simulink model "Chapter7"  (R2024b)
settings: Solver=ode4  StartTime=0.0  StopTime=SIM.StopTime  FixedStep=SIM.FixedStepSize  RelTol=1e-3
values from neighbouring files (symbols this model uses):
  AP = computeAutopilotGains(MAV, TRIM, TFS, DES)    [ch7_main.m]
  CMD = struct()    [ch7_main.m]
  DES = loadDesignParams()    [ch7_main.m]
  LIM = loadSafetyLimits()    [ch7_main.m]
  SNS = loadSensorParameters()    [ch7_main.m]    (also in loadSensorParameters.m = struct())
  TRIM = findTrim(TRIM_MODEL, Va_trim, R_trim, gamma_trim, TRIM_DATA_FILE)    [ch7_main.m]
  WIND = loadWindParameters()    [ch7_main.m]
undefined symbols (not defined in the file or in its folder): DiscIntNeverNeededParam, drawAircraft, F, Light, MAV, MIL, plotter, SIM
libraries: simulink x19, matrix_library x2, aerolibwind2 x1
(part 2 of 2)

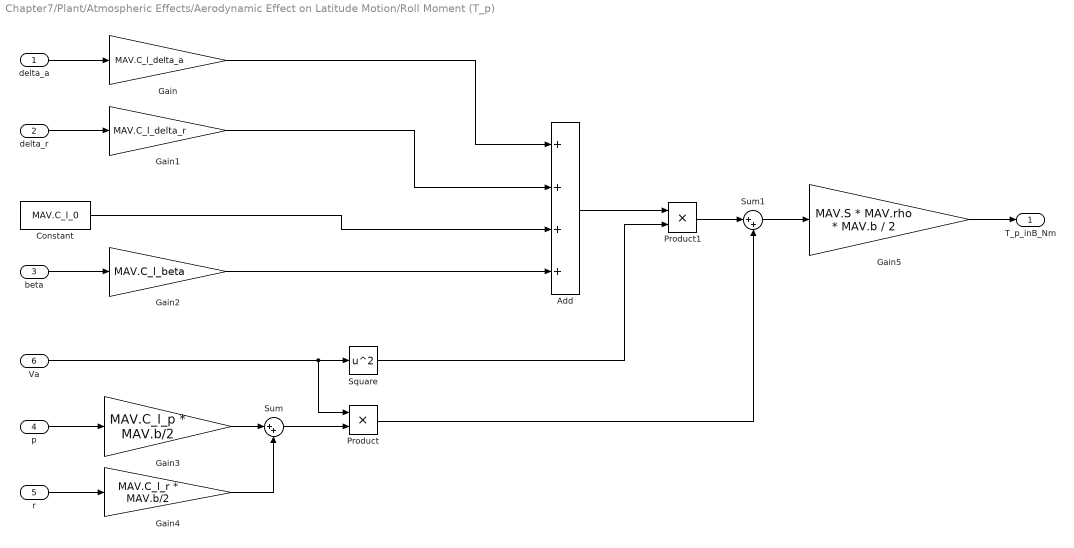
== system Chapter7/Plant/Atmospheric Effects/Aerodynamic Effect on Latitude Motion/Roll Moment (T_p) ==
  delta_a : Inport
  delta_r : Inport  Port=2
  beta : Inport  Port=3
  p : Inport  Port=4
  r : Inport  Port=5
  Va : Inport  Port=6
  Add : Sum  Inputs=++++
  Constant : Constant  Value=MAV.C_l_0
  Gain : Gain  Gain=MAV.C_l_delta_a
  Gain1 : Gain  Gain=MAV.C_l_delta_r
  Gain2 : Gain  Gain=MAV.C_l_beta
  Gain3 : Gain  Gain=MAV.C_l_p * MAV.b/2
  Gain4 : Gain  Gain=MAV.C_l_r * MAV.b/2
  Gain5 : Gain  Gain=MAV.S * MAV.rho * MAV.b / 2
  Product : Product
  Product1 : Product
  Square : Math  Operator=square
  Sum : Sum  Inputs=|++
  Sum1 : Sum  Inputs=|++
  T_p_inB_Nm : Outport
  wires:
  Gain1/1 -> Add/2
  Gain/1 -> Add/1
  Va/1 -> Square/1, Product/1
  Sum/1 -> Product/2
  Gain4/1 -> Sum/2
  Gain3/1 -> Sum/1
  r/1 -> Gain4/1
  p/1 -> Gain3/1
  Gain2/1 -> Add/4
  beta/1 -> Gain2/1
  Constant/1 -> Add/3
  delta_r/1 -> Gain1/1
  delta_a/1 -> Gain/1
  Add/1 -> Product1/1
  Square/1 -> Product1/2
  Product1/1 -> Sum1/1
  Product/1 -> Sum1/2
  Sum1/1 -> Gain5/1
  Gain5/1 -> T_p_inB_Nm/1

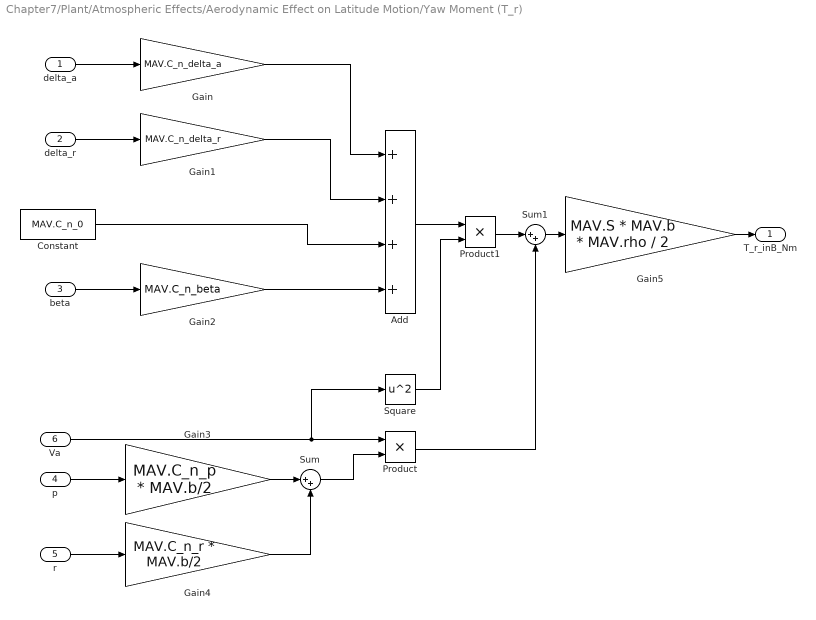
== system Chapter7/Plant/Atmospheric Effects/Aerodynamic Effect on Latitude Motion/Yaw Moment (T_r) ==
  delta_a : Inport
  delta_r : Inport  Port=2
  beta : Inport  Port=3
  p : Inport  Port=4
  r : Inport  Port=5
  Va : Inport  Port=6
  Add : Sum  Inputs=++++
  Constant : Constant  Value=MAV.C_n_0
  Gain : Gain  Gain=MAV.C_n_delta_a
  Gain1 : Gain  Gain=MAV.C_n_delta_r
  Gain2 : Gain  Gain=MAV.C_n_beta
  Gain3 : Gain  Gain=MAV.C_n_p * MAV.b/2
  Gain4 : Gain  Gain=MAV.C_n_r * MAV.b/2
  Gain5 : Gain  Gain=MAV.S * MAV.b * MAV.rho / 2
  Product : Product
  Product1 : Product
  Square : Math  Operator=square
  Sum : Sum  Inputs=|++
  Sum1 : Sum  Inputs=|++
  T_r_inB_Nm : Outport
  wires:
  Gain2/1 -> Add/4
  Constant/1 -> Add/3
  Gain1/1 -> Add/2
  delta_a/1 -> Gain/1
  p/1 -> Gain3/1
  Sum/1 -> Product/2
  Gain/1 -> Add/1
  r/1 -> Gain4/1
  Va/1 -> Square/1, Product/1
  Gain3/1 -> Sum/1
  delta_r/1 -> Gain1/1
  beta/1 -> Gain2/1
  Gain4/1 -> Sum/2
  Add/1 -> Product1/1
  Square/1 -> Product1/2
  Product1/1 -> Sum1/1
  Product/1 -> Sum1/2
  Sum1/1 -> Gain5/1
  Gain5/1 -> T_r_inB_Nm/1

== system Chapter7/Plant/Atmospheric Effects/Aerodynamic Effect on Longitudinal Motion/Drag ==
  delta_e : Inport
  q : Inport  Port=2
  Va : Inport  Port=3
  C_D_of_alpha : Inport  Port=4
  Gain : Gain  Gain=MAV.S * MAV.rho / 2
  Gain2 : Gain  Gain=MAV.C_D_delta_e
  Gain3 : Gain  Gain=MAV.C_D_q * MAV.c / 2
  Product : Product
  Product1 : Product
  Square : Math  Operator=square
  Sum : Sum  Inputs=|++
  Sum1 : Sum  Inputs=|++
  F_Drag_inS_N : Outport
  wires:
  Gain2/1 -> Sum/2
  delta_e/1 -> Gain2/1
  C_D_of_alpha/1 -> Sum/1
  q/1 -> Gain3/1
  Va/1 -> Square/1, Product/1
  Gain3/1 -> Product/2
  Sum/1 -> Product1/1
  Square/1 -> Product1/2
  Product1/1 -> Sum1/1
  Product/1 -> Sum1/2
  Sum1/1 -> Gain/1
  Gain/1 -> F_Drag_inS_N/1

== system Chapter7/Plant/Atmospheric Effects/Aerodynamic Effect on Longitudinal Motion/Lift  ==
  delta_e : Inport
  C_L_of_alpha : Inport  Port=2
  q : Inport  Port=3
  Va : Inport  Port=4
  Gain : Gain  Gain=MAV.C_L_delta_e
  Gain1 : Gain  Gain=MAV.C_L_q * MAV.c / 2
  Gain2 : Gain  Gain=MAV.S * MAV.rho / 2
  Product : Product
  Product1 : Product
  Square : Math  Operator=square
  Sum : Sum  Inputs=|++
  Sum1 : Sum  Inputs=|++
  F_Lift_inS_N : Outport
  wires:
  Gain/1 -> Sum/1
  C_L_of_alpha/1 -> Sum/2
  delta_e/1 -> Gain/1
  q/1 -> Gain1/1
  Gain1/1 -> Product/2
  Va/1 -> Product/1, Square/1
  Sum/1 -> Product1/1
  Square/1 -> Product1/2
  Product1/1 -> Sum1/1
  Product/1 -> Sum1/2
  Sum1/1 -> Gain2/1
  Gain2/1 -> F_Lift_inS_N/1

== system Chapter7/Plant/Atmospheric Effects/Aerodynamic Effect on Longitudinal Motion/Pitch Moment ==
  delta_e : Inport
  alpha : Inport  Port=2
  q : Inport  Port=3
  Va : Inport  Port=4
  Add1 : Sum  Inputs=+++
  Constant : Constant  Value=MAV.C_M_0
  Gain : Gain  Gain=MAV.S * MAV.rho * MAV.c / 2
  Gain1 : Gain  Gain=MAV.C_M_alpha
  Gain2 : Gain  Gain=MAV.C_M_delta_e
  Gain3 : Gain  Gain=MAV.C_M_q * MAV.c / 2
  Product : Product
  Product1 : Product
  Square : Math  Operator=square
  Sum : Sum  Inputs=|++
  T_q_inB_Nm : Outport
  wires:
  delta_e/1 -> Gain2/1
  Gain2/1 -> Add1/1
  alpha/1 -> Gain1/1
  Gain1/1 -> Add1/2
  Constant/1 -> Add1/3
  q/1 -> Gain3/1
  Gain3/1 -> Product/2
  Va/1 -> Product/1, Square/1
  Add1/1 -> Product1/1
  Square/1 -> Product1/2
  Product1/1 -> Sum/1
  Product/1 -> Sum/2
  Sum/1 -> Gain/1
  Gain/1 -> T_q_inB_Nm/1

== system Chapter7/Plant/Atmospheric Effects/Aerodynamic Effect on Longitudinal Motion/Variant Subsystem ==
  note: 1) Add Subsystem or Model blocks as valid variant choices.
      | 2) You cannot connect blocks at this level. At simulation, connectivity is automatically
      | determined, based on the active variant and port name matching.
  alpha : Inport
  Linear Lift Drag Effect of Alpha : Subsystem  VariantControl=LNG_MODEL == 1
  Nonlinear Lift Drag Effect of Alpha : Subsystem  VariantControl=LNG_MODEL == 2
  C_L_of_alpha : Outport
  C_D_of_alpha : Outport  Port=2

== system Chapter7/Plant/Atmospheric Effects/Aerodynamic Effect on Longitudinal Motion/Variant Subsystem/Linear Lift Drag Effect of Alpha ==
  alpha : Inport
  Constant : Constant  Value=MAV.C_L0_
  Constant1 : Constant  Value=MAV.C_D0_
  Gain : Gain  Gain=MAV.C_L_alpha
  Gain1 : Gain  Gain=MAV.C_D_alpha
  Sum : Sum  Inputs=++|
  Sum1 : Sum  Inputs=|++
  C_L_of_alpha : Outport
  C_D_of_alpha : Outport  Port=2
  wires:
  Gain/1 -> Sum/2
  Constant/1 -> Sum/1
  Sum/1 -> C_L_of_alpha/1
  alpha/1 -> Gain1/1, Gain/1
  Gain1/1 -> Sum1/1
  Constant1/1 -> Sum1/2
  Sum1/1 -> C_D_of_alpha/1

== system Chapter7/Plant/Atmospheric Effects/Aerodynamic Effect on Longitudinal Motion/Variant Subsystem/Nonlinear Lift Drag Effect of Alpha ==
  alpha : Inport
  Add : Sum
  Constant : Constant  Value=MAV.C_L0_
  Constant1 : Constant  Value=MAV.C_D_p
  Constant2 : Constant  Value=MAV.C_e * MAV.C_AR*pi
  Divide : Product  Inputs=*/
  Equation 4.10 : MATLAB Function  TreatAsAtomicUnit=on
  Equation 4.11 : Sum  Inputs=++|
  From : From
  Gain : Gain  Gain=MAV.C_L_alpha
  Goto : Goto
  Lift Flat Plate Coefficient Eq 4.8 : Subsystem
  Product : Product
  Product1 : Product
  Square : Math  Operator=square
  Sum : Sum  Inputs=++|
  C_L_of_alpha : Outport
  C_D_of_alpha : Outport  Port=2
  wires:
  Constant/1 -> Sum/1
  alpha/1 -> Lift Flat Plate Coefficient Eq 4.8/1(alpha), Equation 4.10/1(alpha), Gain/1
  Gain/1 -> Sum/2
  Sum/1 -> Goto/1, Product/1
  Equation 4.10/1(lambda1) -> Product/2
  Equation 4.10/2(lambda2) -> Product1/1
  Lift Flat Plate Coefficient Eq 4.8/1(C_L_flat_plate) -> Product1/2
  Product/1 -> Add/1
  Product1/1 -> Add/2
  Add/1 -> C_L_of_alpha/1
  From/1 -> Square/1
  Square/1 -> Divide/1
  Constant2/1 -> Divide/2
  Divide/1 -> Equation 4.11/2
  Constant1/1 -> Equation 4.11/1
  Equation 4.11/1 -> C_D_of_alpha/1

== system Chapter7/Plant/Atmospheric Effects/Aerodynamic Effect on Longitudinal Motion/Variant Subsystem/Nonlinear Lift Drag Effect of Alpha/Lift Flat Plate Coefficient Eq 4.8 ==
  alpha : Inport
  Cos : Trigonometry  Operator=cos
  Gain : Gain  Gain=2
  Product : Product  Inputs=3
  Sign : Signum
  Sin : Trigonometry
  Square : Math  Operator=square
  C_L_flat_plate : Outport
  wires:
  alpha/1 -> Cos/1, Sin/1, Sign/1
  Sin/1 -> Square/1
  Product/1 -> Gain/1
  Cos/1 -> Product/3
  Square/1 -> Product/2
  Sign/1 -> Product/1
  Gain/1 -> C_L_flat_plate/1

== matlab function Chapter7/Plant/Atmospheric Effects/Aerodynamic Effect on Longitudinal Motion/Rot_inXZ_plane ==
  data: alpha input; R_B_S output
function R_B_S = fcn(alpha)
    R_B_S = [-sin(alpha) cos(alpha);
             cos(alpha) sin(alpha)];
end

== matlab function Chapter7/Autopilot/Longitudinal Autopilot/Airspeed Hold Control using Throttle /MATLAB Function ==
  data: u_unsat input; I output; u_sat input; Ki_e input
function I = clampAntiWindup(u_unsat, u_sat, Ki_e)
    is_saturated = (u_unsat ~= u_sat);
    is_same_dir = (u_unsat * Ki_e > 0);

    if (is_saturated && is_same_dir), I = 0;
    else, I = Ki_e;
    end
end

== matlab function Chapter7/Autopilot/Longitudinal Autopilot/MATLAB Function ==
  data: h_cmd input; zone output; h input; DES parameter
function zone = determineZone(h_cmd, h, DES)
    persistent current_zone;
    
    % --- SMART INITIALIZATION ---
    if isempty(current_zone)
        if h < DES.Altitude.Takeoff 
            current_zone = 0; % Take-off
        else
            current_zone = 2; % Hold
        end
    end
    
    err = h_cmd - h;
    enter_threshold = DES.Altitude.Threshold; 
    exit_threshold  = enter_threshold / 2; % Hysteresis
    
    % --- STATE MACHINE ---
    switch current_zone
        
        case 0 % --- TAKE-OFF ZONE ---
            if h > DES.Altitude.Takeoff
                current_zone = 1; % Climb Zone'a geç
            end

        case 1 % --- CLIMB ZONE ---
            if err < exit_threshold
                current_zone = 2; 
            end
            
        case 2 % --- HOLD ZONE --- 
            if err > enter_threshold
                current_zone = 1; % Climb
            elseif err < -enter_threshold
                current_zone = 3; % Descend
            end
            
        case 3 % --- DESCEND ZONE ---
            if err > -exit_threshold
                current_zone = 2; % Hold'a geç
            end
            
        otherwise
            current_zone = 2;
    end
    
    zone = current_zone;
end

== matlab function Chapter7/Subsystem1/GPS/MATLAB Function ==
  data: w_ne_inI_2x1 input; psi input; Va input; meas_Vg output; meas_chi output
function [meas_Vg, meas_chi] = gps_Vg_chi(w_ne_inI_2x1, psi, Va)
    Vn = Va * cos(psi) + w_ne_inI_2x1(1);
    Ve = Va * sin(psi) + w_ne_inI_2x1(2);

    meas_Vg = sqrt(Vn^2 + Ve^2);

    meas_chi = atan2(Ve, Vn);
end

== matlab function Chapter7/Plant/Atmospheric Effects/Aerodynamic Effect on Longitudinal Motion/Variant Subsystem/Nonlinear Lift Drag Effect of Alpha/Equation 4.10 ==
  data: alpha input; lambda1 output; MAV parameter; lambda2 output
function [lambda1, lambda2] = fcn(alpha, MAV)
% Equation 4.9 - 4.10    
exp_m = exp(-MAV.M * (alpha - MAV.alpha_0));
exp_p = exp(MAV.M * (alpha + MAV.alpha_0));
lambda2 = ( 1 + exp_m + exp_p) / ((1 + exp_m)*(1 + exp_p));
lambda1 = 1 - lambda2;
end

== matlab function Chapter7/Plant/Gravitational Force/R_B_I_c3 ==
  data: u input; y output
function y = fcn(u)
    y = zeros(3,1);
    y(1) = -sin(u(2));
    y(2) = cos(u(2)) * sin(u(1));
    y(3) = cos(u(2)) * cos(u(1));
end

== matlab function Chapter7/Plant/Subsystem1/MATLAB Function ==
  data: u input; y output
function y = fcn(u)
    y = wrapToPi(u);

== matlab function Chapter7/Plant/Subsystem1/Subsystem/MATLAB Function ==
  data: u input; y output
function y = fcn(u)
    sphi = sin(u(1));
    cphi = cos(u(1));

    sthe = sin(u(2));
    cthe = cos(u(2));

    scthe = 1 / cthe;
    tthe = scthe * sthe;

    y = [1 sphi * tthe cphi*tthe;
         0 cphi -sphi;
         0 sphi*scthe cphi*scthe];

== matlab function Chapter7/Autopilot/Lateral Autopilot/Sideslip Hold Control Loop/MATLAB Function ==
  data: u_unsat input; I output; u_sat input; Ki_e input
function I = clampAntiWindup(u_unsat, u_sat, Ki_e)
    is_saturated = (u_unsat ~= u_sat);
    is_same_dir = (u_unsat * Ki_e > 0);

    if (is_saturated && is_same_dir), I = 0;
    else, I = Ki_e;
    end
end

== matlab function Chapter7/Autopilot/Lateral Autopilot/Course Hold Control Loop/MATLAB Function ==
  data: u_unsat input; I output; u_sat input; Ki_e input
function I = clampAntiWindup(u_unsat, u_sat, Ki_e)
    is_saturated = (u_unsat ~= u_sat);
    is_same_dir = (u_unsat * Ki_e > 0);

    if (is_saturated && is_same_dir), I = 0;
    else, I = Ki_e;
    end
end

== matlab function Chapter7/Autopilot/Lateral Autopilot/Course Hold Control Loop/Roll Hold Control Loop/MATLAB Function ==
  data: u_unsat input; I output; u_sat input; Ki_e input
function I = clampAntiWindup(u_unsat, u_sat, Ki_e)
    is_saturated = (u_unsat ~= u_sat);
    is_same_dir = (u_unsat * Ki_e > 0);

    if (is_saturated && is_same_dir), I = 0;
    else, I = Ki_e;
    end
end

== matlab function Chapter7/Autopilot/Longitudinal Autopilot/Altitude Hold Control Outer Loop/MATLAB Function ==
  data: u_unsat input; I output; u_sat input; Ki_e input
function I = clampAntiWindup(u_unsat, u_sat, Ki_e)
    is_saturated = (u_unsat ~= u_sat);
    is_same_dir = (u_unsat * Ki_e > 0);

    if (is_saturated && is_same_dir), I = 0;
    else, I = Ki_e;
    end
end

== matlab function Chapter7/Autopilot/Longitudinal Autopilot/Airspeed Hold Control using Pitch Outer Loop/MATLAB Function ==
  data: u_unsat input; I output; u_sat input; Ki_e input
function I = clampAntiWindup(u_unsat, u_sat, Ki_e)
    is_saturated = (u_unsat ~= u_sat);
    is_same_dir = (u_unsat * Ki_e > 0);

    if (is_saturated && is_same_dir), I = 0;
    else, I = Ki_e;
    end
end
